simulink model "QUASI_STATIC_MODEL_SIM"  (R2022a)
settings: Solver=VariableStepAuto  StartTime=0.0  StopTime=1180  MaxStep=0.01  RelTol=1e-3
values from neighbouring files (symbols this model uses):
  Cd = 0.28    [Quasi_Static_Model.m]
  Crr = 0.015    [Quasi_Static_Model.m]
  GR = 7.8    [Quasi_Static_Model.m]
  GVW = (Vm+Md)*g    (= 17559.9)    [Quasi_Static_Model.m]
  M_Eff = Motor(2:16,2:16)    [Quasi_Static_Model.m]
  M_Regen_Eff = Motor_Regen(2:16,2:16)    [Quasi_Static_Model.m]
  M_Regen_Speed = Motor_Regen(2:16,1)    [Quasi_Static_Model.m]
  M_Regen_Torque = Motor_Regen(2:16,17)    [Quasi_Static_Model.m]
  M_Speed = Motor(2:16,1)    [Quasi_Static_Model.m]
  M_Torque = Motor(2:16,17)    [Quasi_Static_Model.m]
  MC_Eff = Motor_C(2:16,2:16)    [Quasi_Static_Model.m]
  MC_Regen_Eff = Motor_C_Regen(2:16,2:16)    [Quasi_Static_Model.m]
  MC_Regen_Speed = Motor_C_Regen(2:16,1)    [Quasi_Static_Model.m]
  MC_Regen_Torque = Motor_C_Regen(2:16,17)    [Quasi_Static_Model.m]
  MC_Speed = Motor_C(2:16,1)    [Quasi_Static_Model.m]
  MC_Torque = Motor_C(2:16,17)    [Quasi_Static_Model.m]
  Md = 80    [Quasi_Static_Model.m]
  Rho = 1.225    [Quasi_Static_Model.m]
  Rw = 0.2032    [Quasi_Static_Model.m]
  T_Eff = 0.85    [Quasi_Static_Model.m]
  theta = 0    [Quasi_Static_Model.m]
  Va = 3.8056    [Quasi_Static_Model.m]
  Vm = 1710    [Quasi_Static_Model.m]
settings Model: Creator=sujee  LastModifiedBy=sujee

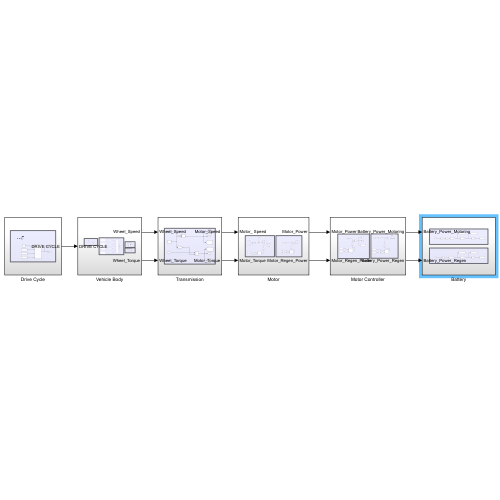
[thumbnail: Simulink's stored preview of the top-level diagram]
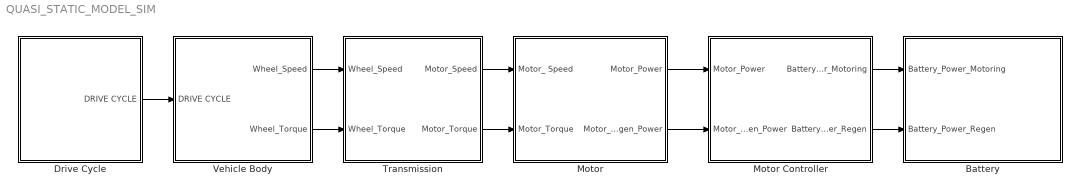
== system QUASI_STATIC_MODEL_SIM ==
  Battery : Subsystem
  Drive Cycle : Subsystem
  Motor : Subsystem
  Motor Controller : Subsystem
  Transmission : Subsystem
  Vehicle Body : Subsystem
  wires:
  Drive Cycle/1(DRIVE CYCLE) -> Vehicle Body/1(DRIVE CYCLE)
  Vehicle Body/1(Wheel_Speed) -> Transmission/1(Wheel_Speed)
  Vehicle Body/2(Wheel_Torque) -> Transmission/2(Wheel_Torque)
  Motor/1(Motor_Power) -> Motor Controller/1(Motor_Power)
  Transmission/1(Motor_Speed) -> Motor/1(Motor_ Speed)
  Transmission/2(Motor_Torque) -> Motor/2(Motor_Torque)
  Motor Controller/1(Battery_Power_Motoring) -> Battery/1(Battery_Power_Motoring)
  Motor/2(Motor_Regen_Power) -> Motor Controller/2(Motor_Regen_Power)
  Motor Controller/2(Battery_Power_Regen) -> Battery/2(Battery_Power_Regen)

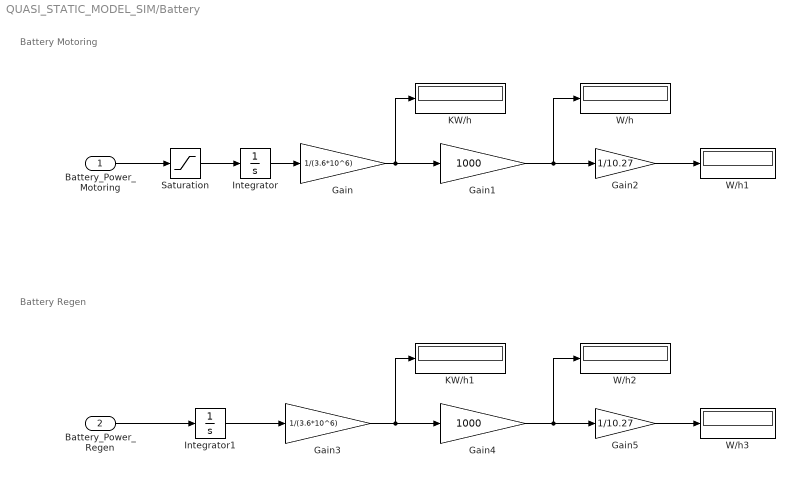
== system QUASI_STATIC_MODEL_SIM/Battery ==
  note: Battery Motoring
  note: Battery Regen
  Battery_Power_Motoring : Inport
  Battery_Power_Regen : Inport  Port=2
  Gain : Gain  Gain=1/(3.6*10^6)
  Gain1 : Gain  Gain=1000
  Gain2 : Gain  Gain=1/10.27
  Gain3 : Gain  Gain=1/(3.6*10^6)
  Gain4 : Gain  Gain=1000
  Gain5 : Gain  Gain=1/10.27
  Integrator : Integrator
  Integrator1 : Integrator
  KW/h : Display
  KW/h1 : Display
  Saturation : Saturate  UpperLimit=inf  LowerLimit=0
  W/h{,1..3} (4 alike) : Display
  wires:
  Battery_Power_Motoring/1 -> Saturation/1
  Saturation/1 -> Integrator/1
  Integrator/1 -> Gain/1
  Gain/1 -> Gain1/1, KW/h/1
  Gain1/1 -> Gain2/1, W/h/1
  Gain2/1 -> W/h1/1
  Gain5/1 -> W/h3/1
  Gain4/1 -> W/h2/1, Gain5/1
  Gain3/1 -> KW/h1/1, Gain4/1
  Integrator1/1 -> Gain3/1
  Battery_Power_Regen/1 -> Integrator1/1

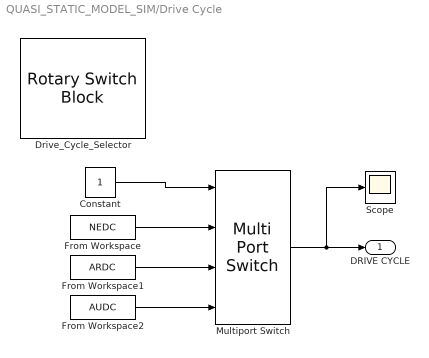
== system QUASI_STATIC_MODEL_SIM/Drive Cycle ==
  Constant : Constant
  Drive_Cycle_Selector : RotarySwitchBlock
      settings: Values={{'NEDC', 'ARDC', 'AUDC'}, [1 2 3]}
  From Workspace : FromWorkspace  VariableName=NEDC
  From Workspace1 : FromWorkspace  VariableName=ARDC
  From Workspace2 : FromWorkspace  VariableName=AUDC
  Multiport Switch : MultiPortSwitch  SaturateOnIntegerOverflow=off  InputSameDT=off
  Scope : Scope
  DRIVE CYCLE : Outport
  wires:
  From Workspace/1 -> Multiport Switch/2
  From Workspace2/1 -> Multiport Switch/4
  From Workspace1/1 -> Multiport Switch/3
  Constant/1 -> Multiport Switch/1
  Multiport Switch/1 -> Scope/1, DRIVE CYCLE/1

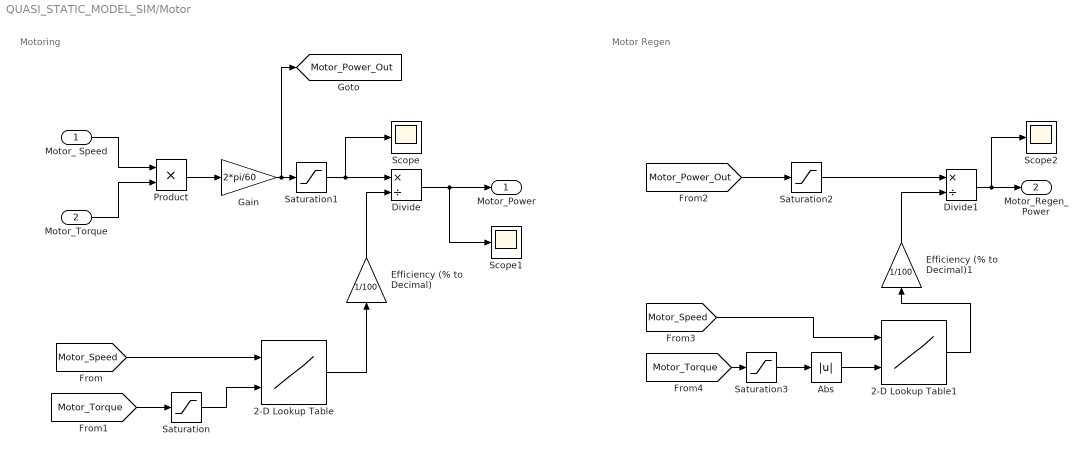
== system QUASI_STATIC_MODEL_SIM/Motor ==
  note: Motor Regen
  note: Motoring
  Motor_ Speed : Inport
  Motor_Torque : Inport  Port=2
  2-D Lookup Table : Lookup_n-D  BreakpointsForDimension1=M_Speed  BreakpointsForDimension2=M_Torque  Table=M_Eff  InternalRulePriority=Speed  RndMeth=Simplest
      settings: InputPortMap=u0,u1
  2-D Lookup Table1 : Lookup_n-D  BreakpointsForDimension1=M_Regen_Speed  BreakpointsForDimension2=M_Regen_Torque  Table=M_Regen_Eff  InternalRulePriority=Speed  RndMeth=Simplest
      settings: InputPortMap=u0,u1
  Abs : Abs  SaturateOnIntegerOverflow=off
  Divide : Product  Inputs=*/
  Divide1 : Product  Inputs=*/
  Efficiency (% to Decimal) : Gain  Gain=1/100
  Efficiency (% to Decimal)1 : Gain  Gain=1/100
  Gain : Gain  Gain=2*pi/60
  Product : Product
  Saturation : Saturate  UpperLimit=inf  LowerLimit=0
  Saturation1 : Saturate  UpperLimit=inf  LowerLimit=0
  Saturation2 : Saturate  UpperLimit=0  LowerLimit=-inf
  Saturation3 : Saturate  UpperLimit=0  LowerLimit=-inf
  Scope : Scope
  Scope1 : Scope
  Scope2 : Scope
  Motor_Power : Outport
  Motor_Regen_Power : Outport  Port=2
  tag scope: Motor_Power_Out=global
  wires:
  Motor_ Speed/1 -> Product/1
  Motor_Torque/1 -> Product/2
  Product/1 -> Gain/1
  Divide/1 -> Scope1/1, Motor_Power/1
  [Motor_Speed] -> 2-D Lookup Table/1
  [Motor_Torque] -> Saturation/1
  Saturation/1 -> 2-D Lookup Table/2
  2-D Lookup Table/1 -> Efficiency (% to Decimal)/1
  Efficiency (% to Decimal)/1 -> Divide/2
  Gain/1 -> [Motor_Power_Out], Saturation1/1
  Saturation1/1 -> Scope/1, Divide/1
  [Motor_Power_Out] -> Saturation2/1
  2-D Lookup Table1/1 -> Efficiency (% to Decimal)1/1
  [Motor_Torque] -> Saturation3/1
  [Motor_Speed] -> 2-D Lookup Table1/1
  Efficiency (% to Decimal)1/1 -> Divide1/2
  Saturation3/1 -> Abs/1
  Abs/1 -> 2-D Lookup Table1/2
  Saturation2/1 -> Divide1/1
  Divide1/1 -> Scope2/1, Motor_Regen_Power/1

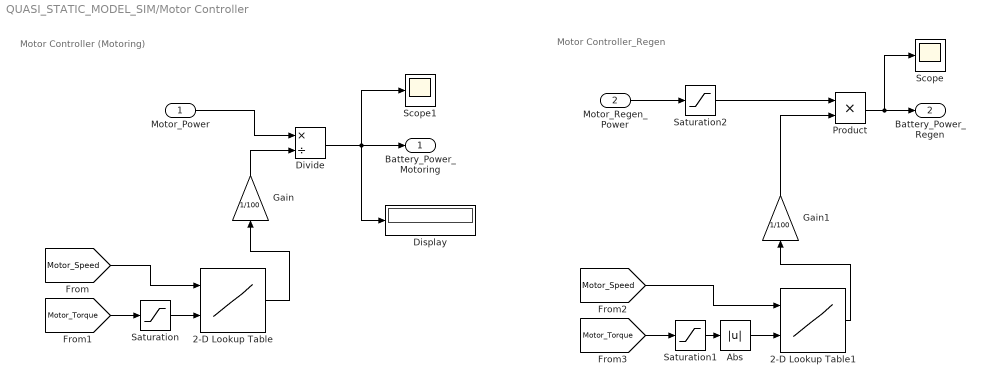
== system QUASI_STATIC_MODEL_SIM/Motor Controller ==
  note: Motor Controller_Regen
  note: Motor Controller (Motoring)
  Motor_Power : Inport
  Motor_Regen_Power : Inport  Port=2
  2-D Lookup Table : Lookup_n-D  BreakpointsForDimension1=MC_Speed  BreakpointsForDimension2=MC_Torque  Table=MC_Eff  InternalRulePriority=Speed  RndMeth=Simplest
      settings: InputPortMap=u0,u1
  2-D Lookup Table1 : Lookup_n-D  BreakpointsForDimension1=MC_Regen_Speed  BreakpointsForDimension2=MC_Regen_Torque  Table=MC_Regen_Eff  InternalRulePriority=Speed  RndMeth=Simplest
      settings: InputPortMap=u0,u1
  Abs : Abs  SaturateOnIntegerOverflow=off
  Display : Display
  Divide : Product  Inputs=*/
  Gain : Gain  Gain=1/100
  Gain1 : Gain  Gain=1/100
  Product : Product
  Saturation : Saturate  UpperLimit=inf  LowerLimit=0
  Saturation1 : Saturate  UpperLimit=0  LowerLimit=-inf
  Saturation2 : Saturate  UpperLimit=0  LowerLimit=-inf
  Scope : Scope
  Scope1 : Scope
  Battery_Power_Motoring : Outport
  Battery_Power_Regen : Outport  Port=2
  wires:
  Motor_Power/1 -> Divide/1
  Divide/1 -> Scope1/1, Display/1, Battery_Power_Motoring/1
  [Motor_Torque] -> Saturation/1
  Saturation/1 -> 2-D Lookup Table/2
  [Motor_Speed] -> 2-D Lookup Table/1
  2-D Lookup Table/1 -> Gain/1
  Gain/1 -> Divide/2
  [Motor_Speed] -> 2-D Lookup Table1/1
  [Motor_Torque] -> Saturation1/1
  2-D Lookup Table1/1 -> Gain1/1
  Motor_Regen_Power/1 -> Saturation2/1
  Saturation1/1 -> Abs/1
  Abs/1 -> 2-D Lookup Table1/2
  Saturation2/1 -> Product/1
  Gain1/1 -> Product/2
  Product/1 -> Scope/1, Battery_Power_Regen/1

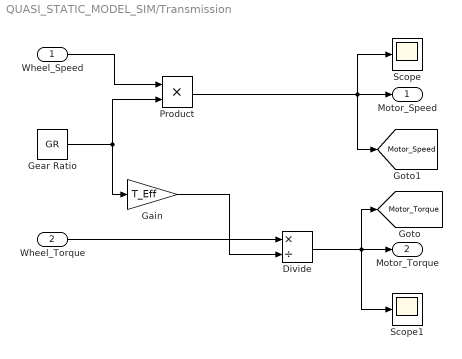
== system QUASI_STATIC_MODEL_SIM/Transmission ==
  Wheel_Speed : Inport
  Wheel_Torque : Inport  Port=2
  Divide : Product  Inputs=*/
  Gain : Gain  Gain=T_Eff
  Gear Ratio : Constant  Value=GR
  Product : Product
  Scope : Scope
  Scope1 : Scope
  Motor_Speed : Outport
  Motor_Torque : Outport  Port=2
  tag scope: Motor_Speed=global, Motor_Torque=global
  wires:
  Gear Ratio/1 -> Product/2, Gain/1
  Wheel_Speed/1 -> Product/1
  Product/1 -> [Motor_Speed], Scope/1, Motor_Speed/1
  Divide/1 -> [Motor_Torque], Scope1/1, Motor_Torque/1
  Gain/1 -> Divide/2
  Wheel_Torque/1 -> Divide/1

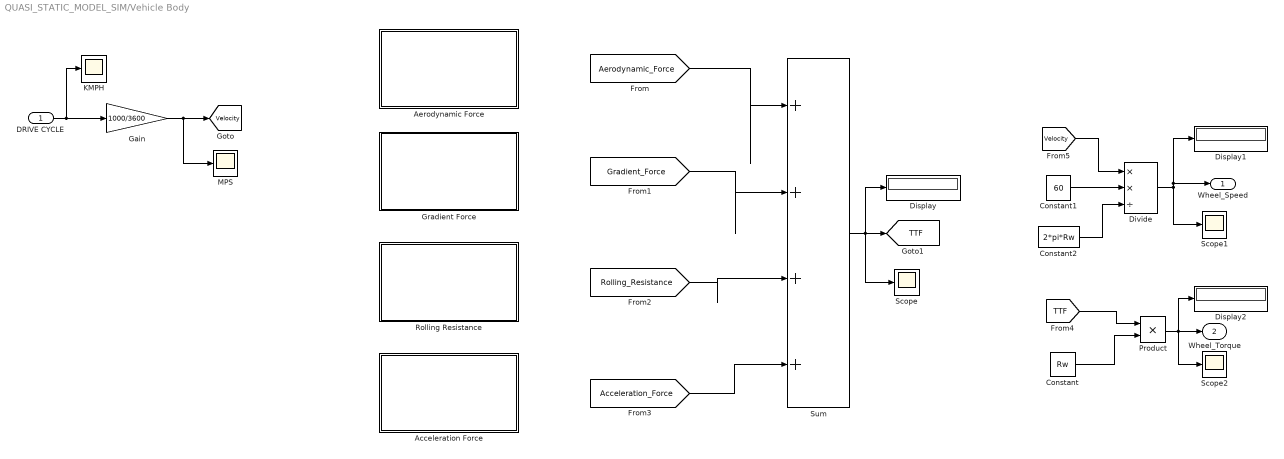
== system QUASI_STATIC_MODEL_SIM/Vehicle Body ==
  DRIVE CYCLE : Inport
  Acceleration Force : Subsystem
  Aerodynamic Force : Subsystem
  Constant : Constant  Value=Rw
  Constant1 : Constant  Value=60
  Constant2 : Constant  Value=2*pi*Rw
  Display : Display
  Display1 : Display
  Display2 : Display
  Divide : Product  Inputs=**/
  Gain : Gain  Gain=1000/3600
  Gradient Force : Subsystem
  KMPH : Scope
  MPS : Scope
  Product : Product
  Rolling Resistance : Subsystem
  Scope : Scope
  Scope1 : Scope
  Scope2 : Scope
  Sum : Sum  Inputs=|++++
  Wheel_Speed : Outport
  Wheel_Torque : Outport  Port=2
  tag scope: TTF=global, Velocity=global
  wires:
  DRIVE CYCLE/1 -> KMPH/1, Gain/1
  Gain/1 -> [Velocity], MPS/1
  [Acceleration_Force] -> Sum/4
  [Rolling_Resistance] -> Sum/3
  [Gradient_Force] -> Sum/2
  [Aerodynamic_Force] -> Sum/1
  Sum/1 -> Display/1, Scope/1, [TTF]
  [TTF] -> Product/1
  Constant/1 -> Product/2
  [Velocity] -> Divide/1
  Constant1/1 -> Divide/2
  Constant2/1 -> Divide/3
  Divide/1 -> Wheel_Speed/1, Display1/1, Scope1/1
  Product/1 -> Wheel_Torque/1, Scope2/1, Display2/1

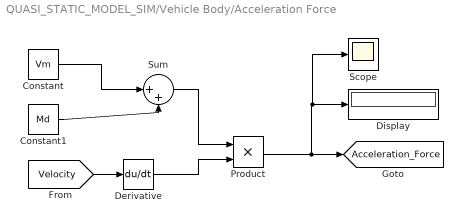
== system QUASI_STATIC_MODEL_SIM/Vehicle Body/Acceleration Force ==
  Constant : Constant  Value=Vm
  Constant1 : Constant  Value=Md
  Derivative : Derivative
  Display : Display
  Product : Product
  Scope : Scope
  Sum : Sum  Inputs=|++
  tag scope: Acceleration_Force=global
  wires:
  Sum/1 -> Product/1
  Derivative/1 -> Product/2
  Product/1 -> Scope/1, Display/1, [Acceleration_Force]
  Constant/1 -> Sum/1
  Constant1/1 -> Sum/2
  [Velocity] -> Derivative/1

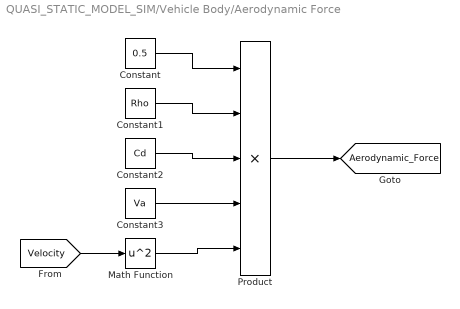
== system QUASI_STATIC_MODEL_SIM/Vehicle Body/Aerodynamic Force ==
  Constant : Constant  Value=0.5
  Constant1 : Constant  Value=Rho
  Constant2 : Constant  Value=Cd
  Constant3 : Constant  Value=Va
  Math Function : Math  Operator=square
  Product : Product  Inputs=5
  tag scope: Aerodynamic_Force=global
  wires:
  [Velocity] -> Math Function/1
  Constant/1 -> Product/1
  Constant1/1 -> Product/2
  Constant2/1 -> Product/3
  Constant3/1 -> Product/4
  Math Function/1 -> Product/5
  Product/1 -> [Aerodynamic_Force]

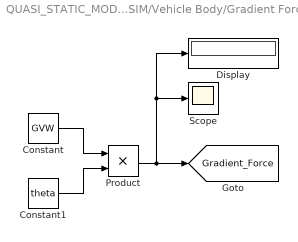
== system QUASI_STATIC_MODEL_SIM/Vehicle Body/Gradient Force ==
  Constant : Constant  Value=GVW
  Constant1 : Constant  Value=theta
  Display : Display
  Product : Product
  Scope : Scope
  tag scope: Gradient_Force=global
  wires:
  Constant/1 -> Product/1
  Constant1/1 -> Product/2
  Product/1 -> Scope/1, Display/1, [Gradient_Force]

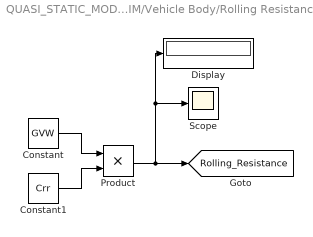
== system QUASI_STATIC_MODEL_SIM/Vehicle Body/Rolling Resistance ==
  Constant : Constant  Value=GVW
  Constant1 : Constant  Value=Crr
  Display : Display
  Product : Product
  Scope : Scope
  tag scope: Rolling_Resistance=global
  wires:
  Constant/1 -> Product/1
  Constant1/1 -> Product/2
  Product/1 -> Display/1, Scope/1, [Rolling_Resistance]
